simulink model "inv_psm"  (R2026b)
settings: Solver=ode23tb  StopTime=param.sim.simlength  FixedStep=param.sim.tc  MaxStep=param.glb_time.tc
values from neighbouring files (symbols this model uses):
  param = struct()    [init_model.m]
undefined symbols (not defined in the file or in its folder): magnitude
libraries: fl_lib x155, nesl_utility x77, igbt_simple_2th_lib x6, lithium_ion_battery x2, simple_flexible_shaft x2, cstblocks_lti x2, dclink_with_center_tap x1, three_phase_pwm_modulator x1, three_phase_inverter_ideal_switch_based_model x1, three_phase_inverter_igbt_advanced_thermal_model x1, three_phase_inverter_mosfet_based_with_thermal_model x1, threephase_inductor_lib x1
(part 2 of 6)

== system inv_psm/inv_psm_mod1/output_filter/threephase_vi_measures_stack ==
  Bus Creator : BusCreator  Inputs=6
  Current Sensor : fl_lib/Electrical/Electrical Sensors/Current Sensor
  Current Sensor1 : fl_lib/Electrical/Electrical Sensors/Current Sensor
  Current Sensor2 : fl_lib/Electrical/Electrical Sensors/Current Sensor
  Gain : Gain  Gain=1/param.psm.machine.ibez
  Gain1 : Gain  Gain=1/param.psm.machine.ibez
  Gain2 : Gain  Gain=1/param.psm.machine.ibez
  Gain3 : Gain  Gain=1/param.psm.machine.ubez
  Gain4 : Gain  Gain=1/param.psm.machine.ubez
  Gain5 : Gain  Gain=1/param.psm.machine.ubez
  Selector : Selector  InputPortWidth=6  IndexOptions=Index vector (dialog)  Indices=[1 2 3]  OutputSizes=1  RuntimeRangeChecks=off
  Selector1 : Selector  InputPortWidth=6  IndexOptions=Index vector (dialog)  Indices=[4 5 6]  OutputSizes=1  RuntimeRangeChecks=off
  Voltage Sensor : fl_lib/Electrical/Electrical Sensors/Voltage Sensor
  Voltage Sensor1 : fl_lib/Electrical/Electrical Sensors/Voltage Sensor
  Voltage Sensor2 : fl_lib/Electrical/Electrical Sensors/Voltage Sensor
  iu_inv : nesl_utility/PS-Simulink Converter  PhysicalDomain=network_engine_domain  SubClassName=ps_output  LeftPortType=input  RightPortType=output  PseudoPeriodic=off  Frequencies=[]  VectorFormat=1-D array  Unit=A  AffineConversion=off
  iv_inv : nesl_utility/PS-Simulink Converter  PhysicalDomain=network_engine_domain  SubClassName=ps_output  LeftPortType=input  RightPortType=output  PseudoPeriodic=off  Frequencies=[]  VectorFormat=1-D array  Unit=A  AffineConversion=off
  iw_inv : nesl_utility/PS-Simulink Converter  PhysicalDomain=network_engine_domain  SubClassName=ps_output  LeftPortType=input  RightPortType=output  PseudoPeriodic=off  Frequencies=[]  VectorFormat=1-D array  Unit=A  AffineConversion=off
  uu_inv : nesl_utility/PS-Simulink Converter  PhysicalDomain=network_engine_domain  SubClassName=ps_output  LeftPortType=input  RightPortType=output  PseudoPeriodic=off  Frequencies=[]  VectorFormat=1-D array  Unit=V  AffineConversion=off
  uv_inv : nesl_utility/PS-Simulink Converter  PhysicalDomain=network_engine_domain  SubClassName=ps_output  LeftPortType=input  RightPortType=output  PseudoPeriodic=off  Frequencies=[]  VectorFormat=1-D array  Unit=V  AffineConversion=off
  uw_inv : nesl_utility/PS-Simulink Converter  PhysicalDomain=network_engine_domain  SubClassName=ps_output  LeftPortType=input  RightPortType=output  PseudoPeriodic=off  Frequencies=[]  VectorFormat=1-D array  Unit=V  AffineConversion=off
  Uu : PMIOPort  Side=Left
  uu : PMIOPort  Port=2  Side=Right
  Uv : PMIOPort  Port=3  Side=Left
  uv : PMIOPort  Port=4  Side=Right
  Uw : PMIOPort  Port=5  Side=Left
  uw : PMIOPort  Port=6  Side=Right
  tag scope: is_uvw_pu_mod1=global, us_uvw_pu_mod1=global
  wires:
  Bus Creator/1 -> Selector/1, Selector1/1  "vi_data"
  Selector/1 -> [us_uvw_pu_mod1]
  iv_inv/1 -> Gain1/1  "iv_inv"
  iu_inv/1 -> Gain/1  "iu_inv"
  iw_inv/1 -> Gain2/1  "iw_inv"
  uu_inv/1 -> Gain3/1  "uu_inv"
  uv_inv/1 -> Gain4/1  "uv_inv"
  uw_inv/1 -> Gain5/1  "uw_inv"
  Selector1/1 -> [is_uvw_pu_mod1]
  Gain/1 -> Bus Creator/4  "iu_inv_pu"
  Gain1/1 -> Bus Creator/5  "iv_inv_pu"
  Gain2/1 -> Bus Creator/6  "iw_inv_pu"
  Gain3/1 -> Bus Creator/1  "uu_inv_pu"
  Gain4/1 -> Bus Creator/2  "uv_inv_pu"
  Gain5/1 -> Bus Creator/3  "uw_inv_pu"
  connections:
  Current Sensor1/LConn1 -- Voltage Sensor1/LConn1 -- Voltage Sensor/RConn2 -- Uv/RConn1
  Voltage Sensor/RConn1 -- uu_inv/LConn1
  Current Sensor/RConn2 -- uu/RConn1
  Voltage Sensor1/RConn1 -- uv_inv/LConn1
  Voltage Sensor2/LConn1 -- Current Sensor2/LConn1 -- Voltage Sensor1/RConn2 -- Uw/RConn1
  Current Sensor/LConn1 -- Voltage Sensor2/RConn2 -- Voltage Sensor/LConn1 -- Uu/RConn1
  Current Sensor1/RConn2 -- uv/RConn1
  Voltage Sensor2/RConn1 -- uw_inv/LConn1
  iv_inv/LConn1 -- Current Sensor1/RConn1
  iu_inv/LConn1 -- Current Sensor/RConn1
  iw_inv/LConn1 -- Current Sensor2/RConn1
  Current Sensor2/RConn2 -- uw/RConn1

== system inv_psm/inv_psm_mod1/inverter/inverter/sv_pwm ==
  gate_cmds_uvw : Inport
  Bus Selector2 : BusSelector  OutputSignals=du(k),dv(k),dw(k)
  Constant1 : Constant  Value=param.inv.behav.pwm_phase_shift_mod1
  modulator1 : Subsystem
  td2tc_1 : TransferFcn  Denominator=[param.glb_time.tc 1]
  td2tc_2 : TransferFcn  Denominator=[param.glb_time.tc 1]
  td2tc_3 : TransferFcn  Denominator=[param.glb_time.tc 1]
  gate_cmds : Outport
  wires:
  modulator1/1(gate_cmds) -> gate_cmds/1
  Constant1/1 -> modulator1/4(phase)
  Bus Selector2/1 -> td2tc_1/1  "<du(k)>"
  Bus Selector2/2 -> td2tc_2/1  "<dv(k)>"
  Bus Selector2/3 -> td2tc_3/1  "<dw(k)>"
  gate_cmds_uvw/1 -> Bus Selector2/1
  td2tc_1/1 -> modulator1/1(u)  "du(t)"
  td2tc_3/1 -> modulator1/3(w)  "dw(t)"
  td2tc_2/1 -> modulator1/2(v)  "dv(t)"

== system inv_psm/inv_psm_mod1/inverter/inverter/three_phase_inverter_ideal_switch_based_model ==
  gate_commands : Inport
  measurements : Subsystem
  three_phase_inverter_ideal_switch_based_model : three_phase_inverter_ideal_switch_based_model/three phase inverter ideal switch based model  Ron_ideal_switch=param.inv.ideal_switch.Rds_on  Vth=param.inv.ideal_switch.Vth  Vgamma=param.inv.ideal_switch.Vdon_diode  Rdon_diode=param.inv.ideal_switch.Rdon_diode  Csnubber=param.inv.ideal_switch.Csnubber  Rsnubber=param.inv.ideal_switch.Rsnubber
  u : PMIOPort  Side=Right
  udc(+) : PMIOPort  Port=2  Side=Left
  v : PMIOPort  Port=3  Side=Right
  udc(-) : PMIOPort  Port=4  Side=Left
  w : PMIOPort  Port=5  Side=Right
  wires:
  three_phase_inverter_ideal_switch_based_model/1 -> measurements/1(m)
  gate_commands/1 -> three_phase_inverter_ideal_switch_based_model/1
  connections:
  three_phase_inverter_ideal_switch_based_model/RConn1 -- u/RConn1
  three_phase_inverter_ideal_switch_based_model/RConn3 -- w/RConn1
  three_phase_inverter_ideal_switch_based_model/RConn2 -- v/RConn1
  three_phase_inverter_ideal_switch_based_model/LConn2 -- udc(-)/RConn1
  three_phase_inverter_ideal_switch_based_model/LConn1 -- udc(+)/RConn1

== system inv_psm/inv_psm_mod1/inverter/inverter/three_phase_inverter_igbt_adv_thermal_model ==
  gate_commands : Inport
  Bus Selector1 : BusSelector  OutputSignals=module_1.igbt_ploss_Q2,module_1.igbt_voltage_Q2,module_1.igbt_current_Q2,module_1.igbt_JH_temp_Q2,module_1.igbt_HA_temp_Q2
  Bus Selector2 : BusSelector  OutputSignals=module_1.igbt_ploss_Q1,module_1.igbt_voltage_Q1,module_1.igbt_current_Q1,module_1.igbt_JH_temp_Q1,module_1.igbt_HA_temp_Q1
  Bus Selector3 : BusSelector  OutputSignals=module_2.igbt_ploss_Q3,module_2.igbt_voltage_Q3,module_2.igbt_current_Q3,module_2.igbt_JH_temp_Q3,module_2.igbt_HA_temp_Q3
  Bus Selector4 : BusSelector  OutputSignals=module_1.diode_ploss_Q1,module_1.diode_JH_temp_Q1,module_1.diode_HA_temp_Q1
  Bus Selector5 : BusSelector  OutputSignals=module_1.diode_ploss_Q2,module_1.diode_JH_temp_Q2,module_1.diode_HA_temp_Q2
  three_phase_inverter_igbt_adv_thermal_model : three_phase_inverter_igbt_advanced_thermal_model/three_phase_inverter_igbt_adv_thermal_model  Commented=on  mass_heatsink_m=param.thermal.heatsink.no_weight  specific_heat_m=param.thermal.heatsink.cp  rth_switch_HA_m=param.thermal.heatsink.Rth_switch_HA  rth_switch_JH_m=param.inv.igbt.Rth_switch_JH  rth_diode_HA_m=param.inv.igbt.Rth_diode_CH  rth_diode_JH_m=param.inv.igbt.Rth_diode_JH  Rce_on_m=param.inv.igbt.Rce_on  Vce_sat_m=param.inv.igbt.Vce_sat  Vth_m=param.inv.igbt.Vth  Eon_m=param.inv.igbt.Eon  Eoff_m=param.inv.igbt.Eoff  Erec_m=param.inv.igbt.Erec  Irr_m=param.inv.igbt.Irr  Voff_sw_loss_m=param.inv.igbt.Voff_sw_losses  Ion_sw_loss_m=param.inv.igbt.Ion_sw_losses  Vdon_diode_m=param.inv.igbt.Vdon_diode  Rdon_diode_m=param.inv.igbt.Rdon_diode  Csnubber_m=param.inv.igbt.Csnubber  Rsnubber_m=param.inv.igbt.Rsnubber  JunctionTermalMass_m=param.inv.igbt.JunctionTermalMass  Tambient_m=param.thermal.heatsink.Tambient  DThs_init_m=param.thermal.heatsink.DThs_init  Lstray_module_m=param.inv.igbt.Lstray_module  Cies_m=param.inv.igbt.Cies  tc_m=param.glb_time.tc
  three_phase_inverter_with_igbt_simple_2th : Subsystem  mask{vce_sat_m=param.inv.igbt.Vce_sat, v_gamma_m=param.inv.igbt.Vdon_diode, Vth_gate_m=param.inv.igbt.Vth, Vth_gate_hyst_m=0.85, Eon_m=param.inv.igbt.Eon*1000, Eoff_m=param.inv.igbt.Eoff*1000, Err_m=param.inv.igbt.Erec*1000, Ic_ref_m=param.inv.igbt.Ion_sw_losses, Vdc_ref_m=param.inv.igbt.Voff_sw_losses, Vblock_Errf_m=50, rce_on_m=param.inv.igbt.Rce_on*1000, rd_on_m=param.inv.igbt.Rdon_diode*1000, Gce_off_m=1e-6, time_constant_edge_m=param.glb_time.tc, time_constant_ploss_m=1e3, Csnubber_m=param.inv.igbt.Csnubber_zvs, Rsnubber_m=param.inv.igbt.Rsnubber_zvs, rth_switch_JH_m=param.inv.igbt.Rth_switch_JH, rth_switch_HA_m=param.thermal.heatsink.Rth_switch_HA, rth_diode_JH_m=param.inv.igbt.Rth_diode_JH, rth_diode_HA_m=param.thermal.heatsink.Rth_diode_HA, JunctionTermalMass_m=param.inv.igbt.JunctionTermalMass, Tambient_m=param.thermal.Tambient, mass_heatsink_m=param.thermal.heatsink.no_weight, specific_heat_m=param.thermal.heatsink.cp}
      mask prompts: vce_sat_m "Collector-emitter on-stage voltage [V]"; v_gamma_m "Diode forward voltage [V]"; Vth_gate_m "Gate-emitter threshold voltage [V]"; Vth_gate_hyst_m "Half hysteresis band for the switching events [V]"; Eon_m "Turn-on energy at Ic_ref, Vdc_ref [mJ]"; Eoff_m "Turn-off energy at Ic_ref, Vdc_ref [mJ]"; Err_m "Reverse recovery energy at Ic_ref, Vdc_ref [mJ]"; Ic_ref_m "Reference current of the energies [A]"; Vdc_ref_m "Reference voltage of the energies [V]"; Vblock_Errf_m "V block Err"; rce_on_m "IGBT on-state series resistance [mOhm]"; rd_on_m "Diode series resistance [mOhm]"; Gce_off_m "Off-state conductance [1/Ohm]"; time_constant_edge_m "Sample&hold time constant (<< on-time) [us]"; time_constant_ploss_m "Loss averaging time constant (2-5 x Tsw) [us]"; Csnubber_m "Csnubber [F]"; Rsnubber_m "Rsnubber [Ohm]"; rth_switch_JH_m "Thermal impedance Junction-heatsink switch [K/W]"; rth_switch_HA_m "Thermal impedance heatsink-ambient switch[K/W]"; rth_diode_JH_m "Thermal impedance Junction-heatsink diode [K/W]"; rth_diode_HA_m "Thermal impedance heatsink-ambient diode [K/W]"; JunctionTermalMass_m "Junction Thermal Mass [J/K]"; Tambient_m "Ambient temperature [degC]"; mass_heatsink_m "Mass heatsink [kg]"; specific_heat_m "Specific heat capacity of the heatsink [J/K/Kg]"
  u : PMIOPort  Side=Right
  udc(+) : PMIOPort  Port=2  Side=Left
  v : PMIOPort  Port=3  Side=Right
  udc(-) : PMIOPort  Port=4  Side=Left
  w : PMIOPort  Port=5  Side=Right
  tag scope: diode_HA_temp_invQ1=global, diode_HA_temp_invQ2=global, diode_JH_temp_invQ1=global, diode_JH_temp_invQ2=global, diode_ploss_invQ1=global, diode_ploss_invQ2=global, igbt_HA_temp_invQ1=global, igbt_HA_temp_invQ2=global, igbt_HA_temp_invQ3=global, igbt_JH_temp_invQ1=global, igbt_JH_temp_invQ2=global, igbt_JH_temp_invQ3=global, igbt_current_invQ1=global, igbt_current_invQ2=global, igbt_current_invQ3=global, igbt_ploss_invQ1=global, igbt_ploss_invQ2=global, igbt_ploss_invQ3=global, igbt_voltage_invQ1=global, igbt_voltage_invQ2=global, igbt_voltage_invQ3=global
  wires:
  Bus Selector3/2 -> [igbt_voltage_invQ3]  "<igbt_voltage_Q3>"
  Bus Selector1/4 -> [igbt_JH_temp_invQ2]  "<igbt_JH_temp_Q2>"
  Bus Selector1/2 -> [igbt_voltage_invQ2]  "<igbt_voltage_Q2>"
  Bus Selector3/4 -> [igbt_JH_temp_invQ3]  "<igbt_JH_temp_Q3>"
  Bus Selector1/3 -> [igbt_current_invQ2]  "<igbt_current_Q2>"
  Bus Selector2/5 -> [igbt_HA_temp_invQ1]  "<igbt_HA_temp_Q1>"
  Bus Selector3/1 -> [igbt_ploss_invQ3]  "<igbt_ploss_Q3>"
  Bus Selector1/5 -> [igbt_HA_temp_invQ2]  "<igbt_HA_temp_Q2>"
  Bus Selector2/2 -> [igbt_voltage_invQ1]  "<igbt_voltage_Q1>"
  Bus Selector2/1 -> [igbt_ploss_invQ1]  "<igbt_ploss_Q1>"
  Bus Selector2/4 -> [igbt_JH_temp_invQ1]  "<igbt_JH_temp_Q1>"
  Bus Selector2/3 -> [igbt_current_invQ1]  "<igbt_current_Q1>"
  Bus Selector3/3 -> [igbt_current_invQ3]  "<igbt_current_Q3>"
  Bus Selector3/5 -> [igbt_HA_temp_invQ3]  "<igbt_HA_temp_Q3>"
  Bus Selector1/1 -> [igbt_ploss_invQ2]  "<igbt_ploss_Q2>"
  gate_commands/1 -> three_phase_inverter_with_igbt_simple_2th/1(gate_commands)
  Bus Selector4/1 -> [diode_ploss_invQ1]  "<diode_ploss_Q1>"
  Bus Selector4/2 -> [diode_JH_temp_invQ1]  "<diode_JH_temp_Q1>"
  Bus Selector4/3 -> [diode_HA_temp_invQ1]  "<diode_HA_temp_Q1>"
  three_phase_inverter_with_igbt_simple_2th/1(m) -> Bus Selector4/1, Bus Selector5/1, Bus Selector3/1, Bus Selector1/1, Bus Selector2/1
  Bus Selector5/3 -> [diode_HA_temp_invQ2]  "<diode_HA_temp_Q2>"
  Bus Selector5/2 -> [diode_JH_temp_invQ2]  "<diode_JH_temp_Q2>"
  Bus Selector5/1 -> [diode_ploss_invQ2]  "<diode_ploss_Q2>"
  connections:
  three_phase_inverter_with_igbt_simple_2th/LConn2 -- udc(-)/RConn1
  three_phase_inverter_with_igbt_simple_2th/RConn1 -- u/RConn1
  three_phase_inverter_with_igbt_simple_2th/RConn2 -- v/RConn1
  three_phase_inverter_with_igbt_simple_2th/LConn1 -- udc(+)/RConn1
  three_phase_inverter_with_igbt_simple_2th/RConn3 -- w/RConn1

== system inv_psm/inv_psm_mod1/inverter/inverter/three_phase_inverter_mosfet_based_with_thermal_model ==
  gate_commands : Inport
  Bus Selector : BusSelector  OutputSignals=mosfet_ploss_Q2,mosfet_voltage_Q2,mosfet_current_Q2,mosfet_JH_temp_Q2,mosfet_HA_temp_Q2
  Bus Selector1 : BusSelector  OutputSignals=mosfet_ploss_Q1,mosfet_voltage_Q1,mosfet_current_Q1,mosfet_JH_temp_Q1,mosfet_HA_temp_Q1
  Bus Selector2 : BusSelector  OutputSignals=mosfet_ploss_Q3,mosfet_voltage_Q3,mosfet_current_Q3,mosfet_JH_temp_Q3,mosfet_HA_temp_Q3
  three phase inverter mosfet based with thermal model : three_phase_inverter_mosfet_based_with_thermal_model/three phase inverter mosfet based with thermal model  mass_heatsink_m=0.2  specific_heat_m=880  rth_mosfet_HA_m=0.02  rth_mosfet_JH_m=0.075  Rds_on_m=0.00185  Vth_m=7.5  Eon_m=0.077  Eoff_m=0.108  Voff_sw_loss_m=1300  Ion_sw_loss_m=1000  Vdon_diode_m=4  Rdon_diode_m=0.00185  JunctionTermalMass_m=2  Tambient_m=40  DThs_init_m=0
  u : PMIOPort  Side=Right
  udc(+) : PMIOPort  Port=2  Side=Left
  v : PMIOPort  Port=3  Side=Right
  udc(-) : PMIOPort  Port=4  Side=Left
  w : PMIOPort  Port=5  Side=Right
  tag scope: mosfet_HA_temp_invQ1=global, mosfet_HA_temp_invQ2=global, mosfet_HA_temp_invQ3=global, mosfet_JH_temp_invQ1=global, mosfet_JH_temp_invQ2=global, mosfet_JH_temp_invQ3=global, mosfet_current_invQ1=global, mosfet_current_invQ2=global, mosfet_current_invQ3=global, mosfet_ploss_invQ1=global, mosfet_ploss_invQ2=global, mosfet_ploss_invQ3=global, mosfet_voltage_invQ1=global, mosfet_voltage_invQ2=global, mosfet_voltage_invQ3=global
  wires:
  gate_commands/1 -> three phase inverter mosfet based with thermal model/1
  three phase inverter mosfet based with thermal model/1 -> Bus Selector/1, Bus Selector2/1, Bus Selector1/1
  Bus Selector2/1 -> [mosfet_ploss_invQ3]  "<mosfet_ploss_Q3>"
  Bus Selector2/2 -> [mosfet_voltage_invQ3]  "<mosfet_voltage_Q3>"
  Bus Selector2/3 -> [mosfet_current_invQ3]  "<mosfet_current_Q3>"
  Bus Selector2/5 -> [mosfet_HA_temp_invQ3]  "<mosfet_HA_temp_Q3>"
  Bus Selector2/4 -> [mosfet_JH_temp_invQ3]  "<mosfet_JH_temp_Q3>"
  Bus Selector/1 -> [mosfet_ploss_invQ2]  "<mosfet_ploss_Q2>"
  Bus Selector/2 -> [mosfet_voltage_invQ2]  "<mosfet_voltage_Q2>"
  Bus Selector/3 -> [mosfet_current_invQ2]  "<mosfet_current_Q2>"
  Bus Selector/4 -> [mosfet_JH_temp_invQ2]  "<mosfet_JH_temp_Q2>"
  Bus Selector/5 -> [mosfet_HA_temp_invQ2]  "<mosfet_HA_temp_Q2>"
  Bus Selector1/1 -> [mosfet_ploss_invQ1]  "<mosfet_ploss_Q1>"
  Bus Selector1/2 -> [mosfet_voltage_invQ1]  "<mosfet_voltage_Q1>"
  Bus Selector1/3 -> [mosfet_current_invQ1]  "<mosfet_current_Q1>"
  Bus Selector1/4 -> [mosfet_JH_temp_invQ1]  "<mosfet_JH_temp_Q1>"
  Bus Selector1/5 -> [mosfet_HA_temp_invQ1]  "<mosfet_HA_temp_Q1>"
  connections:
  three phase inverter mosfet based with thermal model/RConn3 -- w/RConn1
  three phase inverter mosfet based with thermal model/RConn2 -- v/RConn1
  three phase inverter mosfet based with thermal model/LConn1 -- udc(+)/RConn1
  three phase inverter mosfet based with thermal model/LConn2 -- udc(-)/RConn1
  three phase inverter mosfet based with thermal model/RConn1 -- u/RConn1

== system inv_psm/inv_psm_mod1/inverter_ctrl/inverter_control/Speed control ==
  rotor speed : Inport
  rotor speed ref : Inport  Port=2
  1/Ti : Gain  Gain=param.psm.ctrl.kp_w  SaturateOnIntegerOverflow=on  OutDataTypeStr=Inherit: Same as input  ParamDataTypeStr=Inherit: Same as input
  Saturation : Saturate  UpperLimit=param.psm.ctrl.iq_lim  LowerLimit=-param.psm.ctrl.iq_lim
  Sum1 : Sum  Inputs=+++  SaturateOnIntegerOverflow=on
  Sum2 : Sum  Inputs=-+  SaturateOnIntegerOverflow=on
  Sum3 : Sum  Inputs=-+  SaturateOnIntegerOverflow=on
  Unit Delay4 : UnitDelay  SampleTime=-1
  kp : Gain  Gain=param.psm.ctrl.ki_w*param.glb_time.ts_inv  SaturateOnIntegerOverflow=on  OutDataTypeStr=Inherit: Same as input  ParamDataTypeStr=Inherit: Same as input
  torque_ref : Outport
  wires:
  1/Ti/1 -> Sum1/1, Sum3/1
  kp/1 -> Sum1/2
  Sum3/1 -> Unit Delay4/1
  Unit Delay4/1 -> Sum1/3
  rotor speed ref/1 -> Sum2/2
  rotor speed/1 -> Sum2/1
  Sum2/1 -> kp/1, 1/Ti/1
  Sum1/1 -> Saturation/1
  Saturation/1 -> Sum3/2, torque_ref/1

== system inv_psm/inv_psm_mod1/inverter_ctrl/inverter_control/current_ctrl ==
  torque_ref : Inport
  Bus Creator1 : BusCreator  Inputs=2
  bemf_observer : Subsystem
  current_ctrl : Subsystem
  current_transformation : Subsystem
  uab : Outport  VectorParamsAs1DForOutWhenUnconnected=off
  wires:
  [ubeta_pu_mod1] -> Bus Creator1/2  "ub"
  [ualpha_pu_mod1] -> Bus Creator1/1  "ua"
  Bus Creator1/1 -> uab/1
  torque_ref/1 -> current_ctrl/1(iq_ref)  "torque_ref"
  [ibeta_pu_mod1] -> bemf_observer/2(ibeta_pu)
  [ialpha_pu_mod1] -> bemf_observer/1(ialpha_pu)
  [ualpha_pu_mod1] -> bemf_observer/3(ualpha_pu)
  [ubeta_pu_mod1] -> bemf_observer/4(ubeta_pu)
  [udcd_pu_inv_mod1] -> current_ctrl/2(udc_pu), bemf_observer/5(udc_pu)

== system inv_psm/inv_psm_mod1/inverter_ctrl/inverter_control/encoder-sensorless-switch ==
  Constant : Constant  Value=param.psm.ctrl.omega_th
  MATLAB Function : MATLAB Function  TreatAsAtomicUnit=on
  Variant Source1 : VariantSource  VariantControls={param.psm.mode.use_psm_encoder == 1, param.psm.mode.use_psm_encoder == 0}
  Variant Source2 : VariantSource  VariantControls={param.psm.mode.use_psm_encoder == 1, param.psm.mode.use_psm_encoder == 0}
  double_integrator_observer : Subsystem
  omega_pu_psm/hat1 : Scope  NumInputPorts=2
      settings: ActiveDisplayYMinimum=-0.21852300797833357  ActiveDisplayYMaximum=0.24346722517047281  DataLoggingVariableName=ScopeData13
  phase_elec_psm/hat : Scope  NumInputPorts=2
      settings: ActiveDisplayYMinimum=-1  ActiveDisplayYMaximum=1  DataLoggingVariableName=ScopeData12
  tag scope: motor_phase_ctrl_mod1=scoped, motor_speed_pu_ctrl_mod1=scoped
  wires:
  Variant Source1/1 -> [motor_speed_pu_ctrl_mod1]
  Variant Source2/1 -> [motor_phase_ctrl_mod1]
  [phase_hat_mod1] -> phase_elec_psm/hat/1  "theta_hat_mod1"
  [omega_hat_pu_mod1] -> omega_pu_psm/hat1/1  "omega_hat_pu_mod1"
  [phased_psm] -> double_integrator_observer/1(phase_psm)
  MATLAB Function/1(omega_ctrl) -> Variant Source1/2
  MATLAB Function/2(phase_ctrl) -> Variant Source2/2
  double_integrator_observer/1(phase_psm_hat) -> phase_elec_psm/hat/2, Variant Source2/1, MATLAB Function/1(phase_psm)  "phase_psm_hat"
  double_integrator_observer/2(omega_pu_psm_hat) -> Variant Source1/1, omega_pu_psm/hat1/2, MATLAB Function/2(omega_obs)  "omega_pu_psm_hat"
  [phase_hat_mod1] -> MATLAB Function/3(phase_obs)  "theta_hat_mod1"
  [omega_hat_pu_mod1] -> MATLAB Function/4(omega_psm)  "omega_hat_pu_mod1"
  Constant/1 -> MATLAB Function/5(omega_th)

== system inv_psm/inv_psm_mod1/inverter_ctrl/inverter_control/is inv quantizzation and one step delay ==
  is_abc_pu : Inport
  Demux : Demux  Outputs=3
  Mux : Mux  Inputs=3
  is inv quantizzation and one step delay : Subsystem
  isd_abc_pu : Outport
  wires:
  is inv quantizzation and one step delay/2(isd_v_pu) -> Mux/2
  is_abc_pu/1 -> Demux/1
  is inv quantizzation and one step delay/3(isd_w_pu) -> Mux/3
  is inv quantizzation and one step delay/1(isd_u_pu) -> Mux/1
  Demux/1 -> is inv quantizzation and one step delay/1(is_u_pu)
  Mux/1 -> isd_abc_pu/1
  Demux/3 -> is inv quantizzation and one step delay/3(is_w_pu)
  Demux/2 -> is inv quantizzation and one step delay/2(is_v_pu)

== system inv_psm/inv_psm_mod1/inverter_ctrl/inverter_control/measurements ==
  Gain : Gain  Gain=param.psm.machine.psi_bez
  Gain1 : Gain  Gain=param.psm.machine.psi_bez
  To Workspace10 : ToWorkspace  VariableName=id_pu_sim_mod1  SampleTime=-1
      settings: MaxDataPoints=param.glb_time.Ns_inv
  To Workspace11 : ToWorkspace  VariableName=iq_pu_sim_mod1  SampleTime=-1
      settings: MaxDataPoints=param.glb_time.Ns_inv
  To Workspace12 : ToWorkspace  VariableName=uq_pu_sim_mod1  SampleTime=-1
      settings: MaxDataPoints=param.glb_time.Ns_inv
  To Workspace13 : ToWorkspace  VariableName=iq_pu_ref_sim_mod1  SampleTime=-1
      settings: MaxDataPoints=param.glb_time.Ns_inv
  To Workspace14 : ToWorkspace  VariableName=id_pu_ref_sim_mod1  SampleTime=-1
      settings: MaxDataPoints=param.glb_time.Ns_inv
  To Workspace15 : ToWorkspace  VariableName=u_mot_pu_sim_mod1  SampleTime=-1
      settings: MaxDataPoints=param.glb_time.Ns_inv
  To Workspace2 : ToWorkspace  VariableName=ualpha_pu_sim_mod1  SampleTime=-1
      settings: MaxDataPoints=param.glb_time.Ns_inv
  To Workspace3 : ToWorkspace  VariableName=ubeta_pu_sim_mod1  SampleTime=-1
      settings: MaxDataPoints=param.glb_time.Ns_inv
  To Workspace4 : ToWorkspace  VariableName=psi_pu_alpha_hat_sim_mod1  SampleTime=-1
      settings: MaxDataPoints=param.glb_time.Ns_inv
  To Workspace5 : ToWorkspace  VariableName=psi_pu_beta_hat_sim_mod1  SampleTime=-1
      settings: MaxDataPoints=param.glb_time.Ns_inv
  To Workspace6 : ToWorkspace  VariableName=psi_r_alpha_hat_sim_mod1  SampleTime=-1
      settings: MaxDataPoints=param.glb_time.Ns_inv
  To Workspace7 : ToWorkspace  VariableName=ud_pu_sim_mod1  SampleTime=-1
      settings: MaxDataPoints=param.glb_time.Ns_inv
  To Workspace8 : ToWorkspace  VariableName=psi_r_beta_hat_sim_mod1  SampleTime=-1
      settings: MaxDataPoints=param.glb_time.Ns_inv
  wires:
  [psi_r_alpha_pu_hat_mod1] -> Gain/1
  [ualpha_pu_mod1] -> To Workspace2/1  "ualpha_pu_mod1"
  Gain/1 -> To Workspace6/1  "psi_r_alpha_hat"
  [psi_r_alpha_pu_hat_mod1] -> To Workspace4/1  "phi_alpha_pu_hat"
  [ubeta_pu_mod1] -> To Workspace3/1  "ubeta_pu_mod1"
  [psi_r_beta_pu_hat_mod1] -> To Workspace5/1  "phi_beta_pu_hat"
  Gain1/1 -> To Workspace8/1  "psi_r_beta_hat"
  [psi_r_beta_pu_hat_mod1] -> Gain1/1
  [u_mot_pu_mod1] -> To Workspace15/1  "u_mot_pu_mod1"
  [iq_pu_ref_mod1] -> To Workspace13/1  "iq_pu_ref_mod1"
  [ud_pu_mod1] -> To Workspace7/1  "ud_pu_mod1"
  [uq_pu_mod1] -> To Workspace12/1  "uq_pu_mod1"
  [iq_pu_mod1] -> To Workspace11/1  "iq_pu_mod1"
  [id_pu_mod1] -> To Workspace10/1  "id_pu_mod1"
  [id_pu_ref_mod1] -> To Workspace14/1  "id_pu_ref_mod1"

== system inv_psm/inv_psm_mod1/inverter_ctrl/inverter_control/omega_pu ==
  Abs : Abs  SaturateOnIntegerOverflow=off
  flt : Subsystem
  abs(omega_pu) : Outport
  omega_pu : Outport  Port=2
  wires:
  Abs/1 -> flt/1(input)
  [motor_speed_pu_ctrl_mod1] -> Abs/1, omega_pu/1
  flt/1(output) -> abs(omega_pu)/1

== system inv_psm/inv_psm_mod1/inverter_ctrl/inverter_control/phase_acquisition ==
  phase_psm : Inport
  Quantizer : Quantizer  QuantizationInterval=param.meas.adc_quantization
  Unit Delay : UnitDelay  SampleTime=-1
  Zero-Order Hold : ZeroOrderHold  SampleTime=-1
  phased_psm : Outport
  wires:
  Zero-Order Hold/1 -> Quantizer/1
  Unit Delay/1 -> phased_psm/1
  phase_psm/1 -> Zero-Order Hold/1
  Quantizer/1 -> Unit Delay/1

== system inv_psm/inv_psm_mod1/inverter_ctrl/inverter_control/phase_acquisition1 ==
  omega_psm : Inport
  Gain : Gain  Gain=1/param.psm.machine.omega_bez
  Unit Delay : UnitDelay  SampleTime=-1
  Zero-Order Hold : ZeroOrderHold  SampleTime=-1
  omega_pu_psm : Outport
  wires:
  Zero-Order Hold/1 -> Gain/1
  omega_psm/1 -> Zero-Order Hold/1
  Unit Delay/1 -> omega_pu_psm/1
  Gain/1 -> Unit Delay/1

== system inv_psm/inv_psm_mod1/inverter_ctrl/inverter_control/phase_compensation_1 ==
  local_time : Inport
  master_time : Inport  Port=2
  Zero-Order Hold : ZeroOrderHold  SampleTime=-1
  Zero-Order Hold1 : ZeroOrderHold  SampleTime=-1
  alignment_ctrl : Subsystem
  y : Outport
  wires:
  local_time/1 -> Zero-Order Hold/1
  master_time/1 -> Zero-Order Hold1/1
  alignment_ctrl/1(dp) -> y/1
  Zero-Order Hold/1 -> alignment_ctrl/1(local_time)
  Zero-Order Hold1/1 -> alignment_ctrl/2(master_time)

== system inv_psm/inv_psm_mod1/inverter_ctrl/inverter_control/space_vector ==
  uab_out : Inport
  Bus Creator : BusCreator  Inputs=3
  Bus Selector : BusSelector  OutputSignals=da,db,dc
  Bus Selector1 : BusSelector  OutputSignals=ua,ub
  C Caller : CCaller  FunctionName=sv_pwm_process_simulink  PortSpecificationStruct="%)30     .    V @   8    (     @         %    \"     4    !     0         %  0 \"0    $    _    07)G3F%M90  4&]R=$YA;64 4V-O<&4     26YD97@     5'EP90      4VEZ90      27-';&]B86P   X    P    !@    @    $          4    (     0    ,    !         !   P!O=70 #@   #     &    \"     0         !0    @    !     P    $         $  # &]U=  .    .     8    (    !          %    \"     $    &     0         0   ...(+2669 chars)"
  Constant : Constant  Value=param.glb_time.ts_inv
  Constant1 : Constant
  Data Type Conversion1 : DataTypeConversion  OutDataTypeStr=double  SaturateOnIntegerOverflow=off  RndMeth=Floor
  Data Type Conversion15 : DataTypeConversion  OutDataTypeStr=single  SaturateOnIntegerOverflow=off  RndMeth=Floor
  Data Type Conversion16 : DataTypeConversion  OutDataTypeStr=single  SaturateOnIntegerOverflow=off  RndMeth=Floor
  Data Type Conversion17 : DataTypeConversion  OutDataTypeStr=uint32  SaturateOnIntegerOverflow=off  RndMeth=Floor
  Data Type Conversion18 : DataTypeConversion  OutDataTypeStr=single  SaturateOnIntegerOverflow=off  RndMeth=Floor
  Data Type Conversion2 : DataTypeConversion  OutDataTypeStr=double  SaturateOnIntegerOverflow=off  RndMeth=Floor
  Data Type Conversion3 : DataTypeConversion  OutDataTypeStr=double  SaturateOnIntegerOverflow=off  RndMeth=Floor
  Gain1 : Gain  Gain=sqrt(3)/2
  Gain2 : Gain  Gain=sqrt(3)/2
  duvw : Outport
  wires:
  Data Type Conversion15/1 -> C Caller/2
  Bus Selector/2 -> Data Type Conversion2/1  "<db>"
  Data Type Conversion16/1 -> C Caller/3
  Data Type Conversion18/1 -> C Caller/1
  C Caller/1 -> Bus Selector/1
  Bus Creator/1 -> duvw/1
  Data Type Conversion17/1 -> C Caller/4
  Data Type Conversion1/1 -> Bus Creator/1  "du(k)"
  Bus Selector1/2 -> Gain2/1  "<ub>"
  Bus Selector/3 -> Data Type Conversion3/1  "<dc>"
  Bus Selector1/1 -> Gain1/1  "<ua>"
  Data Type Conversion2/1 -> Bus Creator/2  "dv(k)"
  Gain2/1 -> Data Type Conversion15/1
  Bus Selector/1 -> Data Type Conversion1/1  "<da>"
  Gain1/1 -> Data Type Conversion18/1
  Data Type Conversion3/1 -> Bus Creator/3  "dw(k)"
  Constant/1 -> Data Type Conversion16/1
  uab_out/1 -> Bus Selector1/1
  Constant1/1 -> Data Type Conversion17/1

== system inv_psm/inv_psm_mod1/inverter_ctrl/inverter_control/speed_reference_generator ==
  Step : Step  Time=param.psm.mode.time_start_motor_control  FinalValue=param.load.omega_m_sim/param.psm.machine.omega_m_bez
  Step1 : Step  Commented=on  Time=param.sim.simlength/2  FinalValue=-2*param.load.omega_m_sim/param.psm.machine.omega_m_bez
  Sum : Sum  Inputs=|++
  flt : Subsystem
  omega_ref_pu : Outport
  tag scope: omega_ref_pu_mod1=scoped
  wires:
  Step/1 -> Sum/1
  Step1/1 -> Sum/2
  Sum/1 -> flt/1(input)
  flt/1(output) -> [omega_ref_pu_mod1], omega_ref_pu/1

== system inv_psm/inv_psm_mod1/inverter_ctrl/inverter_control/torque_reference ==
  rotor speed : Inport
  1-D Lookup Table : Lookup_n-D  NumberOfTableDimensions=1  BreakpointsForDimension1=param.load.rpm_base  Table=param.load.torque_base  InternalRulePriority=Speed  RndMeth=Simplest
  Gain : Gain  Gain=-param.load.torque_overload_factor
  Gain1 : Gain  Gain=1/param.psm.machine.tau_bez
  Gain2 : Gain  Gain=param.psm.machine.rpm_nom
  torque_ref : Outport
  wires:
  rotor speed/1 -> Gain2/1
  Gain/1 -> torque_ref/1
  Gain1/1 -> Gain/1
  1-D Lookup Table/1 -> Gain1/1
  Gain2/1 -> 1-D Lookup Table/1

== system inv_psm/inv_psm_mod1/inverter_ctrl/inverter_control/udc_acquisition ==
  udc_pu : Inport
  Quantizer : Quantizer  QuantizationInterval=param.meas.adc_quantization
  Unit Delay : UnitDelay  SampleTime=-1
  Zero-Order Hold : ZeroOrderHold  SampleTime=-1
  udcd_pu : Outport
  wires:
  Quantizer/1 -> Unit Delay/1
  udc_pu/1 -> Zero-Order Hold/1
  Unit Delay/1 -> udcd_pu/1
  Zero-Order Hold/1 -> Quantizer/1

== system inv_psm/inv_psm_mod1/inverter/inverter/sv_pwm/modulator1 ==
  u : Inport
  v : Inport  Port=2
  w : Inport  Port=3
  phase : Inport  Port=4
  Bus Creator : BusCreator  Inputs=3
  Three phase two level PWM generator with global TRGO : three_phase_pwm_modulator/Three phase two level PWM generator with global TRGO  f=param.glb_time.fPWM_INV  m_up=0.98  m_low=0.02  dead_time=param.glb_time.dead_time_INV  pos_cmd_gate=15  neg_cmd_gate=-10  polarity=1  tc=param.glb_time.tc  double_sampling=param.glb_time.TRGO_INV_double_update
      link override gate commands/Bus Selector: OutputSignals=du(t)
      link override gate commands/Bus Selector1: OutputSignals=dv(t)
      link override gate commands/Bus Selector2: OutputSignals=dw(t)
  gate_cmds : Outport
  tag scope: TRGO_inv_module_1=global
  wires:
  [time_inv_module_1] -> Three phase two level PWM generator with global TRGO/1
  Bus Creator/1 -> Three phase two level PWM generator with global TRGO/3
  Three phase two level PWM generator with global TRGO/1 -> [TRGO_inv_module_1]
  u/1 -> Bus Creator/1
  v/1 -> Bus Creator/2
  w/1 -> Bus Creator/3
  phase/1 -> Three phase two level PWM generator with global TRGO/2
  Three phase two level PWM generator with global TRGO/2 -> gate_cmds/1

== system inv_psm/inv_psm_mod1/inverter/inverter/three_phase_inverter_ideal_switch_based_model/measurements ==
  m : Inport
  Bus Selector : BusSelector  OutputSignals=voltage_ee_phase_u,voltage_ee_phase_v,voltage_ee_phase_w
  tag scope: inverter_voltage_ee_phase_u=global, inverter_voltage_ee_phase_v=global, inverter_voltage_ee_phase_w=global
  wires:
  Bus Selector/3 -> [inverter_voltage_ee_phase_w]  "<voltage_ee_phase_w>"
  m/1 -> Bus Selector/1
  Bus Selector/2 -> [inverter_voltage_ee_phase_v]  "<voltage_ee_phase_v>"
  Bus Selector/1 -> [inverter_voltage_ee_phase_u]  "<voltage_ee_phase_u>"

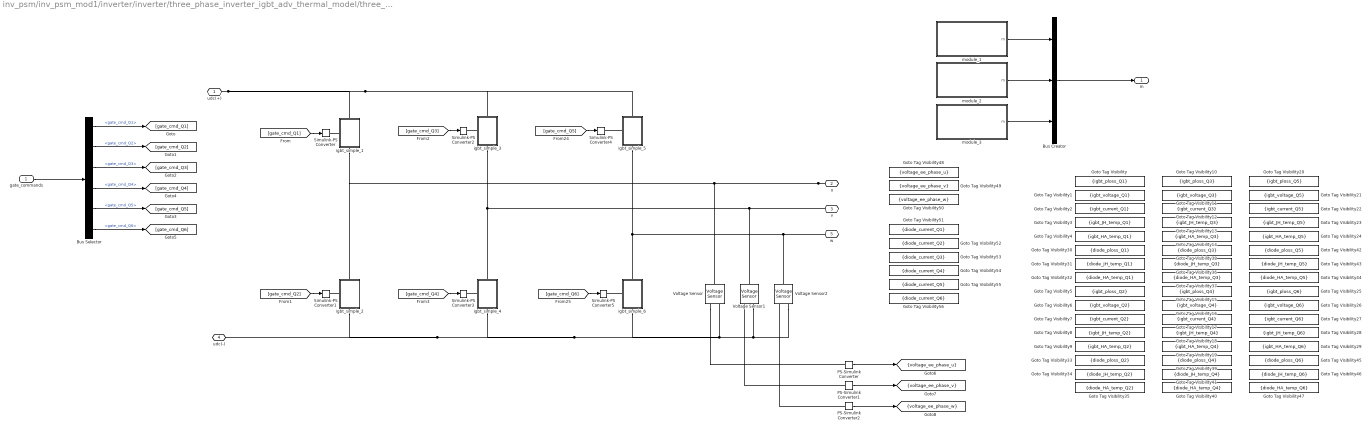
== system inv_psm/inv_psm_mod1/inverter/inverter/three_phase_inverter_igbt_adv_thermal_model/three_phase_inverter_with_igbt_simple_2th ==
  gate_commands : Inport
  Bus Creator : BusCreator  Inputs=3
  Bus Selector : BusSelector  OutputSignals=gate_cmd_Q1,gate_cmd_Q2,gate_cmd_Q3,gate_cmd_Q4,gate_cmd_Q5,gate_cmd_Q6
  Goto Tag Visibility : GotoTagVisibility  GotoTag=igbt_ploss_Q1
  Goto Tag Visibility1 : GotoTagVisibility  GotoTag=igbt_voltage_Q1
  Goto Tag Visibility10 : GotoTagVisibility  GotoTag=igbt_ploss_Q3
  Goto Tag Visibility11 : GotoTagVisibility  GotoTag=igbt_voltage_Q3
  Goto Tag Visibility12 : GotoTagVisibility  GotoTag=igbt_current_Q3
  Goto Tag Visibility13 : GotoTagVisibility  GotoTag=igbt_JH_temp_Q3
  Goto Tag Visibility14 : GotoTagVisibility  GotoTag=igbt_HA_temp_Q3
  Goto Tag Visibility15 : GotoTagVisibility  GotoTag=igbt_ploss_Q4
  Goto Tag Visibility16 : GotoTagVisibility  GotoTag=igbt_voltage_Q4
  Goto Tag Visibility17 : GotoTagVisibility  GotoTag=igbt_current_Q4
  Goto Tag Visibility18 : GotoTagVisibility  GotoTag=igbt_JH_temp_Q4
  Goto Tag Visibility19 : GotoTagVisibility  GotoTag=igbt_HA_temp_Q4
  Goto Tag Visibility2 : GotoTagVisibility  GotoTag=igbt_current_Q1
  Goto Tag Visibility20 : GotoTagVisibility  GotoTag=igbt_ploss_Q5
  Goto Tag Visibility21 : GotoTagVisibility  GotoTag=igbt_voltage_Q5
  Goto Tag Visibility22 : GotoTagVisibility  GotoTag=igbt_current_Q5
  Goto Tag Visibility23 : GotoTagVisibility  GotoTag=igbt_JH_temp_Q5
  Goto Tag Visibility24 : GotoTagVisibility  GotoTag=igbt_HA_temp_Q5
  Goto Tag Visibility25 : GotoTagVisibility  GotoTag=igbt_ploss_Q6
  Goto Tag Visibility26 : GotoTagVisibility  GotoTag=igbt_voltage_Q6
  Goto Tag Visibility27 : GotoTagVisibility  GotoTag=igbt_current_Q6
  Goto Tag Visibility28 : GotoTagVisibility  GotoTag=igbt_JH_temp_Q6
  Goto Tag Visibility29 : GotoTagVisibility  GotoTag=igbt_HA_temp_Q6
  Goto Tag Visibility3 : GotoTagVisibility  GotoTag=igbt_JH_temp_Q1
  Goto Tag Visibility30 : GotoTagVisibility  GotoTag=diode_ploss_Q1
  Goto Tag Visibility31 : GotoTagVisibility  GotoTag=diode_JH_temp_Q1
  Goto Tag Visibility32 : GotoTagVisibility  GotoTag=diode_HA_temp_Q1
  Goto Tag Visibility33 : GotoTagVisibility  GotoTag=diode_ploss_Q2
  Goto Tag Visibility34 : GotoTagVisibility  GotoTag=diode_JH_temp_Q2
  Goto Tag Visibility35 : GotoTagVisibility  GotoTag=diode_HA_temp_Q2
  Goto Tag Visibility36 : GotoTagVisibility  GotoTag=diode_JH_temp_Q3
  Goto Tag Visibility37 : GotoTagVisibility  GotoTag=diode_HA_temp_Q3
  Goto Tag Visibility38 : GotoTagVisibility  GotoTag=diode_ploss_Q3
  Goto Tag Visibility39 : GotoTagVisibility  GotoTag=diode_ploss_Q4
  Goto Tag Visibility4 : GotoTagVisibility  GotoTag=igbt_HA_temp_Q1
  Goto Tag Visibility40 : GotoTagVisibility  GotoTag=diode_HA_temp_Q4
  Goto Tag Visibility41 : GotoTagVisibility  GotoTag=diode_JH_temp_Q4
  Goto Tag Visibility42 : GotoTagVisibility  GotoTag=diode_ploss_Q5
  Goto Tag Visibility43 : GotoTagVisibility  GotoTag=diode_JH_temp_Q5
  Goto Tag Visibility44 : GotoTagVisibility  GotoTag=diode_HA_temp_Q5
  Goto Tag Visibility45 : GotoTagVisibility  GotoTag=diode_ploss_Q6
  Goto Tag Visibility46 : GotoTagVisibility  GotoTag=diode_JH_temp_Q6
  Goto Tag Visibility47 : GotoTagVisibility  GotoTag=diode_HA_temp_Q6
  Goto Tag Visibility48 : GotoTagVisibility  GotoTag=voltage_ee_phase_u
  Goto Tag Visibility49 : GotoTagVisibility  GotoTag=voltage_ee_phase_v
  Goto Tag Visibility5 : GotoTagVisibility  GotoTag=igbt_ploss_Q2
  Goto Tag Visibility50 : GotoTagVisibility  GotoTag=voltage_ee_phase_w
  Goto Tag Visibility51 : GotoTagVisibility  GotoTag=diode_current_Q1
  Goto Tag Visibility52 : GotoTagVisibility  GotoTag=diode_current_Q2
  Goto Tag Visibility53 : GotoTagVisibility  GotoTag=diode_current_Q3
  Goto Tag Visibility54 : GotoTagVisibility  GotoTag=diode_current_Q4
  Goto Tag Visibility55 : GotoTagVisibility  GotoTag=diode_current_Q5
  Goto Tag Visibility56 : GotoTagVisibility  GotoTag=diode_current_Q6
  Goto Tag Visibility6 : GotoTagVisibility  GotoTag=igbt_voltage_Q2
  Goto Tag Visibility7 : GotoTagVisibility  GotoTag=igbt_current_Q2
  Goto Tag Visibility8 : GotoTagVisibility  GotoTag=igbt_JH_temp_Q2
  Goto Tag Visibility9 : GotoTagVisibility  GotoTag=igbt_HA_temp_Q2
  PS-Simulink Converter : nesl_utility/PS-Simulink Converter  PhysicalDomain=network_engine_domain  SubClassName=ps_output  LeftPortType=input  RightPortType=output  PseudoPeriodic=off  Frequencies=[]  VectorFormat=1-D array  Unit=V  AffineConversion=off
  PS-Simulink Converter1 : nesl_utility/PS-Simulink Converter  PhysicalDomain=network_engine_domain  SubClassName=ps_output  LeftPortType=input  RightPortType=output  PseudoPeriodic=off  Frequencies=[]  VectorFormat=1-D array  Unit=V  AffineConversion=off
  PS-Simulink Converter2 : nesl_utility/PS-Simulink Converter  PhysicalDomain=network_engine_domain  SubClassName=ps_output  LeftPortType=input  RightPortType=output  PseudoPeriodic=off  Frequencies=[]  VectorFormat=1-D array  Unit=V  AffineConversion=off
  Simulink-PS Converter{,1..5} (6 alike) : nesl_utility/Simulink-PS Converter  PhysicalDomain=network_engine_domain  SubClassName=ps_input  LeftPortType=input  RightPortType=output  PseudoPeriodic=off  Frequencies=[]  NoiseDistribution=none  NoiseParameters=[]  Unit=V  AffineConversion=off  FilteringAndDerivatives=provide  SimscapeFilterOrder=1  InputFilterTimeConstant=0.001  UdotUserProvided=0
  Voltage Sensor : fl_lib/Electrical/Electrical Sensors/Voltage Sensor
  Voltage Sensor1 : fl_lib/Electrical/Electrical Sensors/Voltage Sensor
  Voltage Sensor2 : fl_lib/Electrical/Electrical Sensors/Voltage Sensor
  igbt_simple_1 : Subsystem
      settings: PortSchema="{\"entries\":[{\"content\":{\"sides\":[{\"content\":{\"connectorIds\":[\"LConn1\"]},\"type\":\"ConnectorPlacement.EquallySpacedRectSide\",\"uuid\":\"9277da8d-d460-43e6-8478-dd662f15d226\"},{\"content\":{\"connectorIds\":[],\"side\":\"RIGHT\"},\"type\":\"ConnectorPlacement.EquallySpacedRectSide\",\"uuid\":\"a7ece396-f1d9-4f4f-a05b-db1fc65d6e1d\"},{\"content\":{\"connectorIds\":[\"LConn2\"],\"side\":\"TOP\"},\"type\":\"ConnectorPlacement.EquallySpacedRectSide\",\"uuid\":\"fdd70777-e9cf-4317-afb6-cae87f75d5b0\"},{\"content\":{\"connectorIds\":[\"RConn1\"],\"side\":\"BOTTOM\"},\"type\":\"ConnectorPlacement.EquallySpacedRectSide\",\"uuid\":\"2353ed68-b1a1-4775-9ca9-31e268d5443b\"}]},\"type\":\"ConnectorPlacement.EquallySpacedConnector\",\"uuid\":\"d5479f4c-4e65-4791-adcb-73df11f88590\"}],\"packageUris\":[\"http://schema.mathworks.com/mf0/Connector/R2020b\"],\"version\":\"1.0\"}"
  igbt_simple_2 : Subsystem
      settings: PortSchema="{\"entries\":[{\"content\":{\"sides\":[{\"content\":{\"connectorIds\":[\"LConn1\"]},\"type\":\"ConnectorPlacement.EquallySpacedRectSide\",\"uuid\":\"9277da8d-d460-43e6-8478-dd662f15d226\"},{\"content\":{\"connectorIds\":[],\"side\":\"RIGHT\"},\"type\":\"ConnectorPlacement.EquallySpacedRectSide\",\"uuid\":\"a7ece396-f1d9-4f4f-a05b-db1fc65d6e1d\"},{\"content\":{\"connectorIds\":[\"LConn2\"],\"side\":\"TOP\"},\"type\":\"ConnectorPlacement.EquallySpacedRectSide\",\"uuid\":\"fdd70777-e9cf-4317-afb6-cae87f75d5b0\"},{\"content\":{\"connectorIds\":[\"RConn1\"],\"side\":\"BOTTOM\"},\"type\":\"ConnectorPlacement.EquallySpacedRectSide\",\"uuid\":\"2353ed68-b1a1-4775-9ca9-31e268d5443b\"}]},\"type\":\"ConnectorPlacement.EquallySpacedConnector\",\"uuid\":\"d5479f4c-4e65-4791-adcb-73df11f88590\"}],\"packageUris\":[\"http://schema.mathworks.com/mf0/Connector/R2020b\"],\"version\":\"1.0\"}"
  igbt_simple_3 : Subsystem
      settings: PortSchema="{\"entries\":[{\"content\":{\"sides\":[{\"content\":{\"connectorIds\":[\"LConn1\"]},\"type\":\"ConnectorPlacement.EquallySpacedRectSide\",\"uuid\":\"9277da8d-d460-43e6-8478-dd662f15d226\"},{\"content\":{\"connectorIds\":[],\"side\":\"RIGHT\"},\"type\":\"ConnectorPlacement.EquallySpacedRectSide\",\"uuid\":\"a7ece396-f1d9-4f4f-a05b-db1fc65d6e1d\"},{\"content\":{\"connectorIds\":[\"LConn2\"],\"side\":\"TOP\"},\"type\":\"ConnectorPlacement.EquallySpacedRectSide\",\"uuid\":\"fdd70777-e9cf-4317-afb6-cae87f75d5b0\"},{\"content\":{\"connectorIds\":[\"RConn1\"],\"side\":\"BOTTOM\"},\"type\":\"ConnectorPlacement.EquallySpacedRectSide\",\"uuid\":\"2353ed68-b1a1-4775-9ca9-31e268d5443b\"}]},\"type\":\"ConnectorPlacement.EquallySpacedConnector\",\"uuid\":\"d5479f4c-4e65-4791-adcb-73df11f88590\"}],\"packageUris\":[\"http://schema.mathworks.com/mf0/Connector/R2020b\"],\"version\":\"1.0\"}"
  igbt_simple_4 : Subsystem
      settings: PortSchema="{\"entries\":[{\"content\":{\"sides\":[{\"content\":{\"connectorIds\":[\"LConn1\"]},\"type\":\"ConnectorPlacement.EquallySpacedRectSide\",\"uuid\":\"9277da8d-d460-43e6-8478-dd662f15d226\"},{\"content\":{\"connectorIds\":[],\"side\":\"RIGHT\"},\"type\":\"ConnectorPlacement.EquallySpacedRectSide\",\"uuid\":\"a7ece396-f1d9-4f4f-a05b-db1fc65d6e1d\"},{\"content\":{\"connectorIds\":[\"LConn2\"],\"side\":\"TOP\"},\"type\":\"ConnectorPlacement.EquallySpacedRectSide\",\"uuid\":\"fdd70777-e9cf-4317-afb6-cae87f75d5b0\"},{\"content\":{\"connectorIds\":[\"RConn1\"],\"side\":\"BOTTOM\"},\"type\":\"ConnectorPlacement.EquallySpacedRectSide\",\"uuid\":\"2353ed68-b1a1-4775-9ca9-31e268d5443b\"}]},\"type\":\"ConnectorPlacement.EquallySpacedConnector\",\"uuid\":\"d5479f4c-4e65-4791-adcb-73df11f88590\"}],\"packageUris\":[\"http://schema.mathworks.com/mf0/Connector/R2020b\"],\"version\":\"1.0\"}"
  igbt_simple_5 : Subsystem
      settings: PortSchema="{\"entries\":[{\"content\":{\"sides\":[{\"content\":{\"connectorIds\":[\"LConn1\"]},\"type\":\"ConnectorPlacement.EquallySpacedRectSide\",\"uuid\":\"9277da8d-d460-43e6-8478-dd662f15d226\"},{\"content\":{\"connectorIds\":[],\"side\":\"RIGHT\"},\"type\":\"ConnectorPlacement.EquallySpacedRectSide\",\"uuid\":\"a7ece396-f1d9-4f4f-a05b-db1fc65d6e1d\"},{\"content\":{\"connectorIds\":[\"LConn2\"],\"side\":\"TOP\"},\"type\":\"ConnectorPlacement.EquallySpacedRectSide\",\"uuid\":\"fdd70777-e9cf-4317-afb6-cae87f75d5b0\"},{\"content\":{\"connectorIds\":[\"RConn1\"],\"side\":\"BOTTOM\"},\"type\":\"ConnectorPlacement.EquallySpacedRectSide\",\"uuid\":\"2353ed68-b1a1-4775-9ca9-31e268d5443b\"}]},\"type\":\"ConnectorPlacement.EquallySpacedConnector\",\"uuid\":\"d5479f4c-4e65-4791-adcb-73df11f88590\"}],\"packageUris\":[\"http://schema.mathworks.com/mf0/Connector/R2020b\"],\"version\":\"1.0\"}"
  igbt_simple_6 : Subsystem
      settings: PortSchema="{\"entries\":[{\"content\":{\"sides\":[{\"content\":{\"connectorIds\":[\"LConn1\"]},\"type\":\"ConnectorPlacement.EquallySpacedRectSide\",\"uuid\":\"9277da8d-d460-43e6-8478-dd662f15d226\"},{\"content\":{\"connectorIds\":[],\"side\":\"RIGHT\"},\"type\":\"ConnectorPlacement.EquallySpacedRectSide\",\"uuid\":\"a7ece396-f1d9-4f4f-a05b-db1fc65d6e1d\"},{\"content\":{\"connectorIds\":[\"LConn2\"],\"side\":\"TOP\"},\"type\":\"ConnectorPlacement.EquallySpacedRectSide\",\"uuid\":\"fdd70777-e9cf-4317-afb6-cae87f75d5b0\"},{\"content\":{\"connectorIds\":[\"RConn1\"],\"side\":\"BOTTOM\"},\"type\":\"ConnectorPlacement.EquallySpacedRectSide\",\"uuid\":\"2353ed68-b1a1-4775-9ca9-31e268d5443b\"}]},\"type\":\"ConnectorPlacement.EquallySpacedConnector\",\"uuid\":\"d5479f4c-4e65-4791-adcb-73df11f88590\"}],\"packageUris\":[\"http://schema.mathworks.com/mf0/Connector/R2020b\"],\"version\":\"1.0\"}"
  module_1 : Subsystem
  module_2 : Subsystem
  module_3 : Subsystem
  udc(+) : PMIOPort  Side=Left
  u : PMIOPort  Port=2  Side=Right
  v : PMIOPort  Port=3  Side=Right
  udc(-) : PMIOPort  Port=4  Side=Left
  w : PMIOPort  Port=5  Side=Right
  m : Outport
  tag scope: voltage_ee_phase_u=scoped, voltage_ee_phase_v=scoped, voltage_ee_phase_w=scoped
  wires:
  module_3/1(m) -> Bus Creator/3
  module_1/1(m) -> Bus Creator/1
  Bus Creator/1 -> m/1
  module_2/1(m) -> Bus Creator/2
  PS-Simulink Converter2/1 -> [voltage_ee_phase_w]
  PS-Simulink Converter1/1 -> [voltage_ee_phase_v]
  PS-Simulink Converter/1 -> [voltage_ee_phase_u]
  Bus Selector/6 -> [gate_cmd_Q6]  "<gate_cmd_Q6>"
  Bus Selector/5 -> [gate_cmd_Q5]  "<gate_cmd_Q5>"
  [gate_cmd_Q6] -> Simulink-PS Converter5/1
  [gate_cmd_Q5] -> Simulink-PS Converter4/1
  [gate_cmd_Q3] -> Simulink-PS Converter2/1
  Bus Selector/2 -> [gate_cmd_Q2]  "<gate_cmd_Q2>"
  Bus Selector/1 -> [gate_cmd_Q1]  "<gate_cmd_Q1>"
  Bus Selector/3 -> [gate_cmd_Q3]  "<gate_cmd_Q3>"
  [gate_cmd_Q4] -> Simulink-PS Converter3/1
  [gate_cmd_Q2] -> Simulink-PS Converter1/1
  [gate_cmd_Q1] -> Simulink-PS Converter/1
  Bus Selector/4 -> [gate_cmd_Q4]  "<gate_cmd_Q4>"
  gate_commands/1 -> Bus Selector/1
  connections:
  PS-Simulink Converter2/LConn1 -- Voltage Sensor2/RConn1
  PS-Simulink Converter1/LConn1 -- Voltage Sensor1/RConn1
  Voltage Sensor/RConn1 -- PS-Simulink Converter/LConn1
  w/RConn1 -- Voltage Sensor2/LConn1 -- igbt_simple_6/LConn2 -- igbt_simple_5/RConn1
  v/RConn1 -- Voltage Sensor1/LConn1 -- igbt_simple_4/LConn2 -- igbt_simple_3/RConn1
  Voltage Sensor1/RConn2 -- Voltage Sensor2/RConn2 -- Voltage Sensor/RConn2 -- igbt_simple_6/RConn1 -- igbt_simple_4/RConn1 -- igbt_simple_2/RConn1 -- udc(-)/RConn1
  igbt_simple_6/LConn1 -- Simulink-PS Converter5/RConn1
  igbt_simple_5/LConn1 -- Simulink-PS Converter4/RConn1
  igbt_simple_4/LConn1 -- Simulink-PS Converter3/RConn1
  igbt_simple_3/LConn1 -- Simulink-PS Converter2/RConn1
  igbt_simple_2/LConn1 -- Simulink-PS Converter1/RConn1
  igbt_simple_1/LConn1 -- Simulink-PS Converter/RConn1
  udc(+)/RConn1 -- igbt_simple_1/LConn2 -- igbt_simple_5/LConn2 -- igbt_simple_3/LConn2
  u/RConn1 -- Voltage Sensor/LConn1 -- igbt_simple_2/LConn2 -- igbt_simple_1/RConn1

== system inv_psm/inv_psm_mod1/inverter_ctrl/inverter_control/current_ctrl/bemf_observer ==
  ialpha_pu : Inport
  ibeta_pu : Inport  Port=2
  ualpha_pu : Inport  Port=3
  ubeta_pu : Inport  Port=4
  udc_pu : Inport  Port=5
  EKF_bemf_observer : Subsystem
  Mux : Mux
  Mux1 : Mux
  Observer Comparison mod1 : Scope  NumInputPorts=2
      settings: ActiveDisplayYMinimum=-4.6842825562218753  ActiveDisplayYMaximum=27.314839860320347
  Variant Source1 : VariantSource  VariantControls={param.psm.impl.use_ekf_bemf_module_1 == 1, param.psm.impl.use_observer_from_simulink_module_1 == 1, param.psm.impl.use_observer_from_ccaller_module_1 == 1}
  Variant Source2 : VariantSource  VariantControls={param.psm.impl.use_ekf_bemf_module_1 == 1, param.psm.impl.use_observer_from_simulink_module_1 == 1, param.psm.impl.use_observer_from_ccaller_module_1 == 1}
  bemf_observer : Subsystem
  bemf_observer_ccaller : Subsystem
  tag scope: omega_hat_pu_mod1=scoped, phase_hat_mod1=scoped
  wires:
  ialpha_pu/1 -> bemf_observer_ccaller/1(ialpha_pu), bemf_observer/1(ialpha_pu), EKF_bemf_observer/1(ialpha_pu)
  ibeta_pu/1 -> bemf_observer_ccaller/2(ibeta_pu), bemf_observer/2(ibeta_pu), EKF_bemf_observer/2(ibeta_pu)
  Mux/1 -> Observer Comparison mod1/1
  Mux1/1 -> Observer Comparison mod1/2
  ualpha_pu/1 -> bemf_observer_ccaller/3(ualpha_pu), bemf_observer/3(ualpha_pu), EKF_bemf_observer/3(ualpha_pu)
  ubeta_pu/1 -> bemf_observer_ccaller/4(ubeta_pu), bemf_observer/4(ubeta_pu), EKF_bemf_observer/4(ubeta_pu)
  Variant Source1/1 -> [phase_hat_mod1]
  Variant Source2/1 -> [omega_hat_pu_mod1]
  udc_pu/1 -> bemf_observer_ccaller/5(udc_pu), bemf_observer/5(udc_pu), EKF_bemf_observer/5(udc_pu)
  [omegad_pu_psm] -> Mux/4  "omega_pu_psm"
  [phased_psm] -> Mux1/4  "phase_psm"
  EKF_bemf_observer/2(omega_elec_ekf_hat) -> [omega_elec_ekf_hat]  "omega_elec_ekf_hat"
  EKF_bemf_observer/1(phase_elec_ekf_hat) -> [phase_elec_ekf_hat]  "phase_elec_ekf_hat"
  bemf_observer/1(omega_pu) -> [omega_elec_bemf_hat]  "omega_elec_bemf_hat"
  bemf_observer/2(theta_hat) -> [phase_elec_bemf_hat]  "phase_elec_bemf_hat"
  bemf_observer_ccaller/2(theta_hat) -> [phase_elec_bemf_cc_hat]  "phase_elec_bemf_cc_hat"
  bemf_observer_ccaller/1(omega_pu) -> [omega_elec_bemf_cc_hat]  "omega_elec_bemf_cc_hat"
  [phase_elec_bemf_cc_hat] -> Mux1/3  "phase_bemf_cc_hat"
  [omega_elec_bemf_cc_hat] -> Mux/3  "omega_bemf_cc_hat"
  [omega_elec_bemf_hat] -> Mux/2  "omega_bemf_hat"
  [phase_elec_bemf_hat] -> Mux1/2  "phase_bemf_hat"
  [phase_elec_ekf_hat] -> Mux1/1  "phase_ekf_hat"
  [omega_elec_ekf_hat] -> Mux/1  "omega_ekf_hat"
  [omega_elec_ekf_hat] -> Variant Source2/1
  [omega_elec_bemf_hat] -> Variant Source2/2
  [omega_elec_bemf_cc_hat] -> Variant Source2/3
  [phase_elec_ekf_hat] -> Variant Source1/1
  [phase_elec_bemf_hat] -> Variant Source1/2
  [phase_elec_bemf_cc_hat] -> Variant Source1/3
